simulink subsystem "DDSRF"  (R2022b)
settings: Solver=VariableStepAuto  StartTime=0.0  StopTime=10.0  RelTol=1e-3
model mask{f_n=50, T_s=1e-4}
  mask prompts: f_n "Nominal frequency [Hz]"; T_s "Sample time [s]"
undefined symbols (not defined in the file or in its folder): alpha
libraries: eeTransforms x2
settings Model: Creator=winkens  LastModifiedBy=winkens
settings SolverCC: AlgebraicLoopSolver=TrustRegion
settings DebuggingCC: UnconnectedInputMsg=warning  UnconnectedOutputMsg=warning  UnconnectedLineMsg=warning  SFMachineParentedDataDiag=warning
settings ModelReferenceCC: EnableRefExpFcnMdlSchedulingChecks=on
settings RTWCC: DLArmComputeVersion=19.05

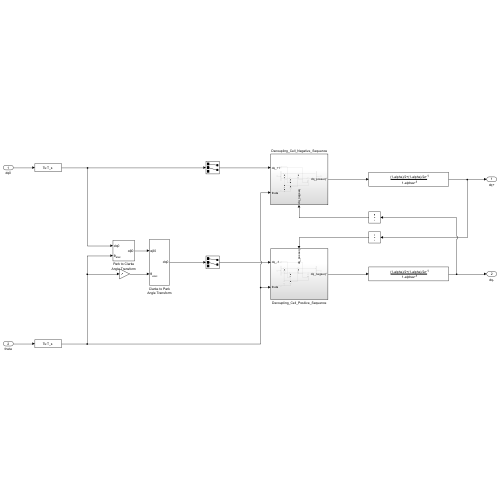
[thumbnail: Simulink's stored preview of the top-level diagram]
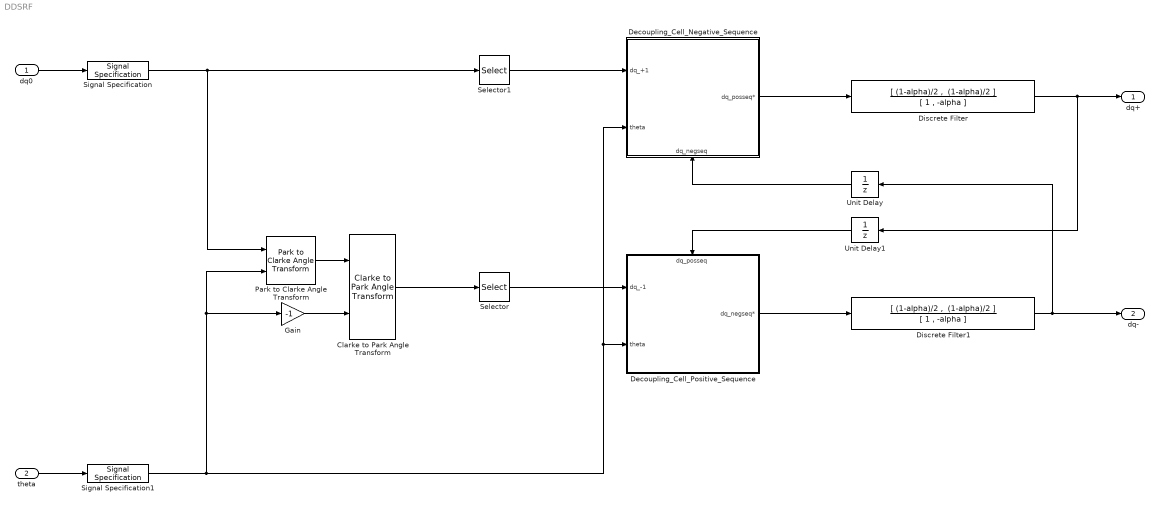
== system DDSRF ==
  dq0 : Inport
  theta : Inport  Port=2
  Clarke to Park Angle Transform : eeTransforms/Clarke to Park Angle Transform  AxisAlignment=D-axis
  Decoupling_Cell_Negative_Sequence : Subsystem
      settings: PortSchema="{\"entries\":[{\"content\":{\"sides\":[{\"content\":{\"connectorIds\":[\"In1\",\"In2\"]},\"type\":\"ConnectorPlacement.EquallySpacedRectSide\",\"uuid\":\"7e4d9097-d147-45b9-a27e-534e9e46aab2\"},{\"content\":{\"connectorIds\":[\"Out1\"],\"side\":\"RIGHT\"},\"type\":\"ConnectorPlacement.EquallySpacedRectSide\",\"uuid\":\"d4fe3eca-d090-48f9-b5c8-e3fbbef2e5d3\"},{\"content\":{\"connectorIds\":[],\"side\":\"TOP\"},\"type\":\"ConnectorPlacement.EquallySpacedRectSide\",\"uuid\":\"da857eb9-490e-4482-a0a7-eca1b9b42d95\"},{\"content\":{\"connectorIds\":[\"In3\"],\"side\":\"BOTTOM\"},\"type\":\"ConnectorPlacement.EquallySpacedRectSide\",\"uuid\":\"37ea14cd-d2b9-432e-8808-e464d0b07519\"},{\"content\":{\"connectorIds\":[],\"side\":\"HIDDEN\"},\"type\":\"ConnectorPlacement.EquallySpacedRectSide\",\"uuid\":\"8fbf3f88-4af7-4787-ba24-005450d8e6de\"}]},\"type\":\"ConnectorPlacement.EquallySpacedConnector\",\"uuid\":\"d0045c60-6cfe-4caf-a9dd-50c25b74b953\"}],\"packageUris\":[\"http://schema.mathworks.com/mf0/Connector/R2020b\"],\"version\":\"1.0\"}"
  Decoupling_Cell_Positive_Sequence : Subsystem
      settings: PortSchema="{\"entries\":[{\"content\":{\"sides\":[{\"content\":{\"connectorIds\":[\"In1\",\"In2\"]},\"type\":\"ConnectorPlacement.EquallySpacedRectSide\",\"uuid\":\"7e4d9097-d147-45b9-a27e-534e9e46aab2\"},{\"content\":{\"connectorIds\":[\"Out1\"],\"side\":\"RIGHT\"},\"type\":\"ConnectorPlacement.EquallySpacedRectSide\",\"uuid\":\"d4fe3eca-d090-48f9-b5c8-e3fbbef2e5d3\"},{\"content\":{\"connectorIds\":[\"In3\"],\"side\":\"TOP\"},\"type\":\"ConnectorPlacement.EquallySpacedRectSide\",\"uuid\":\"da857eb9-490e-4482-a0a7-eca1b9b42d95\"},{\"content\":{\"connectorIds\":[],\"side\":\"BOTTOM\"},\"type\":\"ConnectorPlacement.EquallySpacedRectSide\",\"uuid\":\"37ea14cd-d2b9-432e-8808-e464d0b07519\"},{\"content\":{\"connectorIds\":[],\"side\":\"HIDDEN\"},\"type\":\"ConnectorPlacement.EquallySpacedRectSide\",\"uuid\":\"8fbf3f88-4af7-4787-ba24-005450d8e6de\"}]},\"type\":\"ConnectorPlacement.EquallySpacedConnector\",\"uuid\":\"d0045c60-6cfe-4caf-a9dd-50c25b74b953\"}],\"packageUris\":[\"http://schema.mathworks.com/mf0/Connector/R2020b\"],\"version\":\"1.0\"}"
  Discrete Filter : DiscreteFilter  Numerator="[ (1-alpha)/2 ,  (1-alpha)/2 ]"  Denominator=[ 1 , -alpha ]  SampleTime=T_s
  Discrete Filter1 : DiscreteFilter  Numerator="[ (1-alpha)/2 ,  (1-alpha)/2 ]"  Denominator=[ 1 , -alpha ]  SampleTime=T_s
  Gain : Gain  Gain=-1
  Park to Clarke Angle Transform : eeTransforms/Park to Clarke Angle Transform  AxisAlignment=D-axis
  Selector : Selector  InputPortWidth=3  IndexOptions=Index vector (dialog)  Indices=[1 2]  OutputSizes=1
  Selector1 : Selector  InputPortWidth=3  IndexOptions=Index vector (dialog)  Indices=[1 2]  OutputSizes=1
  Signal Specification : SignalSpecification  SampleTime=T_s
  Signal Specification1 : SignalSpecification  SampleTime=T_s
  Unit Delay : UnitDelay  SampleTime=T_s  HasFrameUpgradeWarning=on
  Unit Delay1 : UnitDelay  SampleTime=T_s  HasFrameUpgradeWarning=on
  dq+ : Outport
  dq- : Outport  Port=2
  wires:
  Park to Clarke Angle Transform/1 -> Clarke to Park Angle Transform/1
  theta/1 -> Signal Specification1/1
  Gain/1 -> Clarke to Park Angle Transform/2
  dq0/1 -> Signal Specification/1
  Clarke to Park Angle Transform/1 -> Selector/1
  Selector1/1 -> Decoupling_Cell_Negative_Sequence/1(dq_+1)
  Selector/1 -> Decoupling_Cell_Positive_Sequence/1(dq_-1)
  Decoupling_Cell_Negative_Sequence/1(dq_posseq*) -> Discrete Filter/1
  Discrete Filter/1 -> Unit Delay1/1, dq+/1
  Decoupling_Cell_Positive_Sequence/1(dq_negseq*) -> Discrete Filter1/1
  Discrete Filter1/1 -> dq-/1, Unit Delay/1
  Signal Specification/1 -> Selector1/1, Park to Clarke Angle Transform/1
  Signal Specification1/1 -> Park to Clarke Angle Transform/2, Gain/1, Decoupling_Cell_Negative_Sequence/2(theta), Decoupling_Cell_Positive_Sequence/2(theta)
  Unit Delay/1 -> Decoupling_Cell_Negative_Sequence/3(dq_negseq)
  Unit Delay1/1 -> Decoupling_Cell_Positive_Sequence/3(dq_posseq)

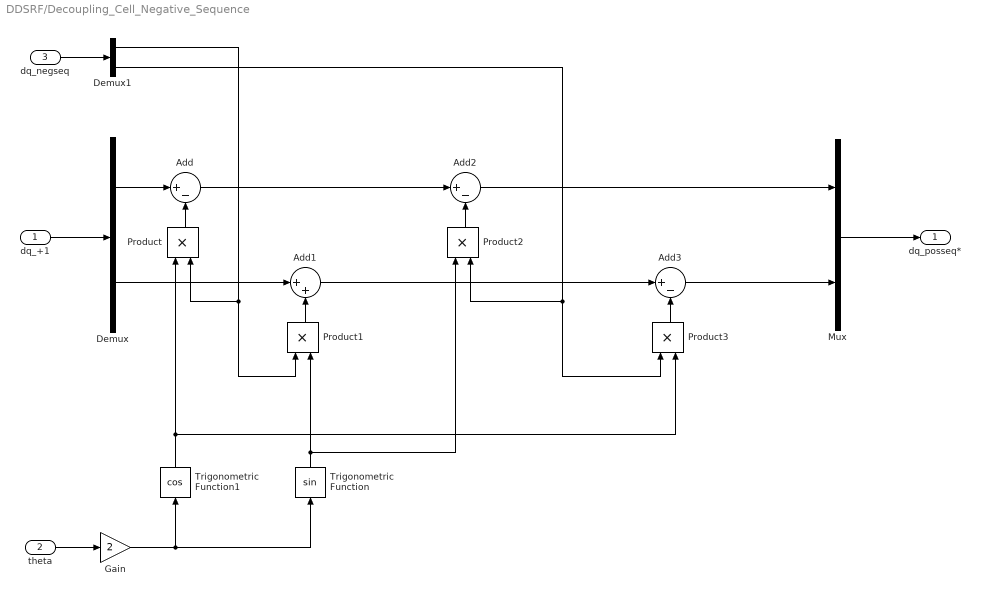
== system DDSRF/Decoupling_Cell_Negative_Sequence ==
  dq_+1 : Inport
  theta : Inport  Port=2
  dq_negseq : Inport  Port=3
  Add : Sum  Inputs=|+-
  Add1 : Sum  Inputs=|++
  Add2 : Sum  Inputs=|+-
  Add3 : Sum  Inputs=|+-
  Demux : Demux  Outputs=2
  Demux1 : Demux  Outputs=2
  Gain : Gain  Gain=2
  Mux : Mux  Inputs=2
  Product{,1..3} (4 alike) : Product
  Trigonometric Function : Trigonometry
  Trigonometric Function1 : Trigonometry  Operator=cos
  dq_posseq* : Outport
  wires:
  dq_+1/1 -> Demux/1
  Demux/1 -> Add/1
  Demux/2 -> Add1/1
  theta/1 -> Gain/1
  Gain/1 -> Trigonometric Function/1, Trigonometric Function1/1
  Product/1 -> Add/2
  Trigonometric Function1/1 -> Product3/2, Product/1
  Product1/1 -> Add1/2
  Trigonometric Function/1 -> Product2/1, Product1/2
  Add/1 -> Add2/1
  Product2/1 -> Add2/2
  Add1/1 -> Add3/1
  Product3/1 -> Add3/2
  dq_negseq/1 -> Demux1/1
  Add3/1 -> Mux/2
  Add2/1 -> Mux/1
  Mux/1 -> dq_posseq*/1
  Demux1/1 -> Product1/1, Product/2
  Demux1/2 -> Product3/1, Product2/2

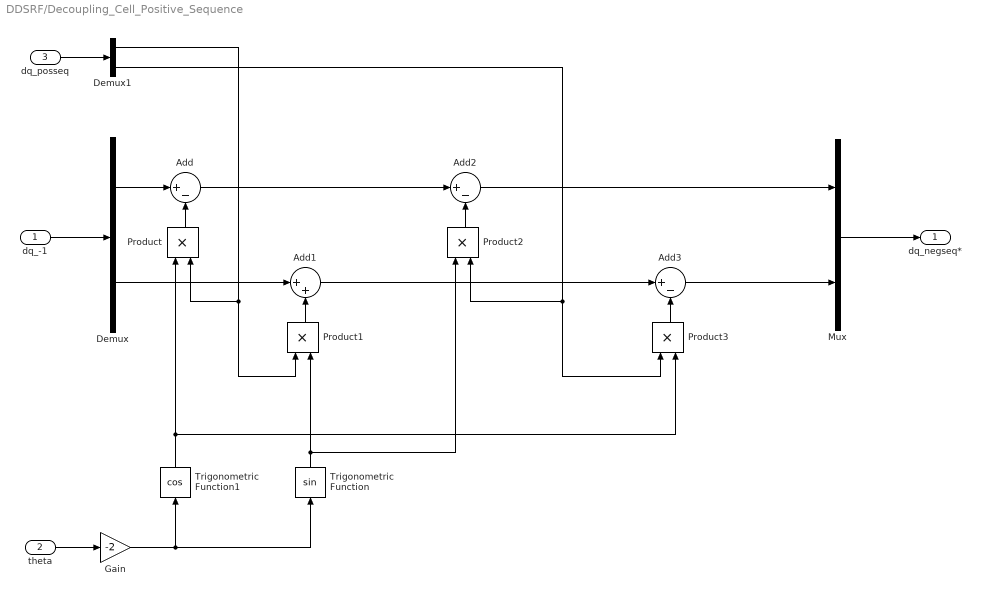
== system DDSRF/Decoupling_Cell_Positive_Sequence ==
  dq_-1 : Inport
  theta : Inport  Port=2
  dq_posseq : Inport  Port=3
  Add : Sum  Inputs=|+-
  Add1 : Sum  Inputs=|++
  Add2 : Sum  Inputs=|+-
  Add3 : Sum  Inputs=|+-
  Demux : Demux  Outputs=2
  Demux1 : Demux  Outputs=2
  Gain : Gain  Gain=-2
  Mux : Mux  Inputs=2
  Product{,1..3} (4 alike) : Product
  Trigonometric Function : Trigonometry
  Trigonometric Function1 : Trigonometry  Operator=cos
  dq_negseq* : Outport
  wires:
  dq_-1/1 -> Demux/1
  Demux/1 -> Add/1
  Demux/2 -> Add1/1
  theta/1 -> Gain/1
  Gain/1 -> Trigonometric Function/1, Trigonometric Function1/1
  Product/1 -> Add/2
  Trigonometric Function1/1 -> Product3/2, Product/1
  Product1/1 -> Add1/2
  Trigonometric Function/1 -> Product2/1, Product1/2
  Add/1 -> Add2/1
  Product2/1 -> Add2/2
  Add1/1 -> Add3/1
  Product3/1 -> Add3/2
  dq_posseq/1 -> Demux1/1
  Add3/1 -> Mux/2
  Add2/1 -> Mux/1
  Mux/1 -> dq_negseq*/1
  Demux1/1 -> Product1/1, Product/2
  Demux1/2 -> Product3/1, Product2/2
